simulink model "Template_v5_0_0_2026a_Original"  (R2026a)
settings: Solver=ode4  StopTime=tsim  FixedStep=baseRate  RelTol=1e-6  AbsTol=1e-6
undefined symbols (not defined in the file or in its folder): baseRate, dataRate, DiscIntNeverNeededParam, F_thrusters_BLACK, F_thrusters_BLUE, F_thrusters_RED, home_states_BLACK, home_states_BLUE, home_states_RED, IBLACK, IBLUE, init_states_BLACK, init_states_BLUE, init_states_RED, IRED, K_BLACK, K_BLUE, K_RED, labConsoleIP, mBLACK, mBLUE, mRED, Phase0_End, Phase1_End, Phase2_End, Phase3_End, Phase3_SubPhase1_End, Phase3_SubPhase2_End, Phase3_SubPhase3_End, Phase3_SubPhase4_End, Phase4_End, Phase5_End, platformSelection, PWMFreq, serverRate, simMode, tableDamping_BLACK, tableDamping_BLUE, tableDamping_RED, tableSlope, thrust_decay_BLACK, thrust_decay_BLUE, thrust_decay_RED, thruster_dist2CG_BLACK, thruster_dist2CG_BLUE, thruster_dist2CG_RED, xLength, yLength
libraries: simulink x18, dspinverses x3, nvidiaCommlib x1
(part 7 of 7)

== matlab function Template_v5_0_0_2026a_Original/Thruster & Float Control Code/Change BLUE Behavior/Calculate Duty Cycle/MATLAB Function5 ==
  data: H_final output; u_desired input; duty_cycles output; x0 input; thruster_dist2CG_BLUE parameter; F_thrusters_BLUE parameter; max_iters parameter; tol parameter; thrust_decay_BLUE parameter
function [H_final, duty_cycles] = optimize_duty_cycle_with_decay( ...
    u_desired, x0, thruster_dist2CG_BLUE, F_thrusters_BLUE, max_iters, tol, thrust_decay_BLUE)
    %OPTIMIZE_DUTY_CYCLE_WITH_DECAY 
    %   Iteratively optimizes thruster duty cycles while updating thrust decay.
    %
    %   Inputs:
    %       u_desired           - Desired force/torque vector [Fx; Fy; M] (3x1)
    %       x0                  - Initial guess for duty cycles (8x1)
    %       thruster_dist2CG_BLUE- Distances of thrusters from CG (vector, mm)
    %       F_thrusters_BLUE     - Thrust of each thruster (8x1, N): calibrated
    %                             (Calibration tab) or nominal (all eight alike)
    %       max_iters           - Maximum optimization iterations
    %       tol                 - Convergence tolerance (on duty cycles)
    %       thrust_decay_BLUE    - Thrust lost per extra valve open at once: with n
    %                             open, each gives 1 - thrust_decay_BLUE*(n - 1) of
    %                             its thrust alone (thruster calibration, Together)
    %
    %   Outputs:
    %       H_final     - Final H-matrix including thrust decay (3x8)
    %       duty_cycles - Optimized duty cycles (8x1)
    %

    % ---------------------------
    % Initialization
    % ---------------------------
    num_thrusters      = length(x0); %#ok<NASGU> % reserved if needed later
    duty_cycles        = x0;                     % current solution
    thrust_decay_factor = ones(8, 1);            % initial decay (each thruster's share)
    prev_duty_cycles   = duty_cycles + 2*tol;    % force first iteration

    % ---------------------------
    % Iterative optimization
    % ---------------------------
    for iter = 1:max_iters
        % Build system matrix H with current decay factor
        H = MakeHWithDecay(thruster_dist2CG_BLUE, F_thrusters_BLUE, thrust_decay_factor);

        % Solve constrained least squares (box constraints: 0 ≤ x ≤ 1)
        duty_cycles = custom_constrained_least_squares(H, u_desired, duty_cycles);

        % Update each thruster's decay from the current duty cycles
        [thrust_decay_factor, ~] = check_thrust_decay(duty_cycles, thrust_decay_BLUE);

        % Check convergence (∞-norm difference)
        if norm(duty_cycles - prev_duty_cycles, Inf) < tol
            H_final = MakeHWithDecayRecalculateForce(thruster_dist2CG_BLUE, F_thrusters_BLUE, thrust_decay_factor);
            return;
        end

        % Update reference for next iteration
        prev_duty_cycles = duty_cycles;
    end

    % If not converged within max_iters, return final H with last decay
    H_final = MakeHWithDecayRecalculateForce(thruster_dist2CG_BLUE, F_thrusters_BLUE, thrust_decay_factor);
end


% ========================================================================
% Custom Constrained Least Squares Solver
% ========================================================================
function x_opt = custom_constrained_least_squares(H, b, x0)
    %CUSTOM_CONSTRAINED_LEAST_SQUARES
    %   Solves min_x ||H*x - b||^2 subject to 0 <= x <= 1
    %   using projected gradient descent with backtracking line search.
    %
    %   Inputs:
    %       H   - System matrix (3x8)
    %       b   - Desired vector (3x1)
    %       x0  - Initial guess (8x1)
    %
    %   Output:
    %       x_opt - Optimal duty cycle vector (8x1)

    % Parameters
    max_iterations = 100;
    tolerance      = 1e-6;
    alpha          = 0.01;  % initial step size
    beta           = 0.5;   % backtracking factor

    % Initialization
    x      = x0;
    x_prev = x0 + 2*tolerance;

    % Precompute matrices
    HtH = H' * H;
    Htb = H' * b;

    for iter = 1:max_iterations
        % Gradient of ||H*x - b||^2
        gradient = 2 * (HtH*x - Htb);

        % Store objective for comparison
        current_obj = norm(H*x - b)^2;

        % Backtracking line search
        step_size = alpha;
        for ls_iter = 1:20
            x_new = x - step_size * gradient;
            x_new = max(0, min(1, x_new)); % project into [0,1]

            new_obj = norm(H*x_new - b)^2;
            if new_obj < current_obj
                break; % accept step
            else
                step_size = step_size * beta;
            end
        end

        % Update
        x = x_new;

        % Convergence check
        if norm(x - x_prev) < tolerance
            break;
        end

        % Adaptive step size tuning
        if iter > 1 && new_obj < current_obj
            alpha = min(alpha * 1.1, 0.1); % speed up if progress
        else
            alpha = alpha * 0.9;           % slow down otherwise
        end

        % Store for next iteration
        x_prev = x;
    end

    x_opt = x;
end


% ========================================================================
% Construct H-matrix (with decay factor)
% ========================================================================
function H = MakeHWithDecay(thruster_dist2CG, F_thrusters, thrust_decay_factor)
    %MAKEHWITHDECAY
    %   Builds the H matrix that maps thruster duty cycles to [Fx; Fy; M],
    %   applying each thruster's thrust decay (8x1, or one for all).
    %
    %   Outputs H as (3x8)

    % Convert thruster arm distances to meters
    adjusted_dist = thruster_dist2CG / 1000;

    % Thruster directions (X, Y, and moment arm)
    Vec1 = [-1; -1;  0;  0;  1;  1;  0;  0]; % X
    Vec2 = [ 0;  0;  1;  1;  0;  0; -1; -1]; % Y
    Vec3 = adjusted_dist;                    % moment (Z)

    Mat1 = [Vec1, Vec2, Vec3]';

    % Thruster forces (scaled by decay)
    F_decayed = F_thrusters(:) .* thrust_decay_factor(:);

    % Build diagonal scaling
    Mat2 = diag(F_decayed / 2);

    % Final mapping
    H = Mat1 * Mat2;
end


% ========================================================================
% Construct H-matrix (recalculate full force with decay)
% ========================================================================
function H = MakeHWithDecayRecalculateForce(thruster_dist2CG, F_thrusters, thrust_decay_factor)
    %MAKEHWITHDECAYRECALCULATEFORCE
    %   Same as MakeHWithDecay but applies full nominal force scaling.

    adjusted_dist = thruster_dist2CG / 1000;

    Vec1 = [-1; -1;  0;  0;  1;  1;  0;  0];
    Vec2 = [ 0;  0;  1;  1;  0;  0; -1; -1];
    Vec3 = adjusted_dist;

    Mat1 = [Vec1, Vec2, Vec3]';

    F_decayed = F_thrusters(:) .* thrust_decay_factor(:);

    Mat2 = diag(F_decayed);

    H = Mat1 * Mat2;
end


% ========================================================================
% Thrust Decay Update Rule
% ========================================================================
function [thrust_decay_factor, count] = check_thrust_decay(PWMs, decay_per_valve)
    %CHECK_THRUST_DECAY
    %   Each thruster's share of its thrust alone over one PWM period. The
    %   valves share one regulated supply: with n open at once, each gives
    %   max(0, 1 - decay_per_valve*(n - 1)) of its thrust alone (linear, as
    %   the thruster calibration's Together stage measures it). The Teensy
    %   opens every valve at the start of each PWM period and closes each
    %   after its duty cycle, so between two closings the number open is
    %   known, and each thruster's share is the average over its own opening.
    %
    %   Inputs:
    %       PWMs            - Duty cycle vector (8x1)
    %       decay_per_valve - Thrust lost per extra valve open (scalar)
    %
    %   Outputs:
    %       thrust_decay_factor - Each thruster's share of its thrust (8x1)
    %       count               - Number of active thrusters

    % Normalize if needed
    if max(PWMs) > 1
        PWMs = PWMs / max(PWMs);
    end
    duty = max(PWMs(:), 0);

    % Active thrusters
    count = sum(duty > 0);

    % The instants the valves close, in order
    closing = sort(duty);

    thrust_decay_factor = ones(8, 1);
    for i = 1:8
        if duty(i) > 0
            share = 0;
            t0 = 0;
            for k = 1:8
                t1 = min(closing(k), duty(i));
                if t1 > t0
                    n_open = sum(duty >= t1);   % valves open from t0 to t1
                    share = share + (t1 - t0) * max(0, 1 - decay_per_valve*(n_open - 1));
                    t0 = t1;
                end
            end
            thrust_decay_factor(i) = share / duty(i);
        end
    end
end

== matlab function Template_v5_0_0_2026a_Original/Thruster & Float Control Code/Change BLUE Behavior/Calculate Duty Cycle/MATLAB Function1 ==
  data: ThrustPer_Final output; ThrustPer input; PWMFreq parameter
function ThrustPer_Final  = ThrusterSat(ThrustPer, PWMFreq)

    ValveTime       = 0.007;
    TControl        = 1/PWMFreq;

    ThrustPer_Final = zeros(8,1);
    
    if max(ThrustPer) > 1
        ThrustPer_Sat = ThrustPer/max(ThrustPer);
    else
        ThrustPer_Sat = ThrustPer;
    end
    
    for i = 1:8
        if ThrustPer_Sat(i) > ValveTime/TControl 
            ThrustPer_Final(i) = ThrustPer_Sat(i);
        else
            ThrustPer_Final(i) = 0;
        end
    end


end

== matlab function Template_v5_0_0_2026a_Original/PhaseSpace Camera Code/Use Hardware to Obtain States/Store RED Data/Subsystem2/Enabled Subsystem/MATLAB Function ==
  data: y input; dy output; dt input; tau input; ema_prev input; ema output
function [dy, ema] = realtime_derivative_ema(y, dt, tau, ema_prev)
    % Compute smoothed derivative using Exponential Moving Average
    %
    % Inputs:
    %   y        : Current measurement
    %   dt       : Time step
    %   tau      : Time constant for EMA filter (larger = more smoothing)
    %   ema_prev : Previous EMA value
    %
    % Outputs:
    %   dy  : Smoothed derivative estimate
    %   ema : Updated EMA value
    
    % Calculate smoothing factor from time constant
    alpha = 1 - exp(-dt ./ tau);
    
    % Update Exponential Moving Average
    ema = alpha .* y + (1 - alpha) .* ema_prev;
    
    % Compute derivative using finite difference on smoothed values
    dy = (ema - ema_prev) ./ dt;
end

== matlab function Template_v5_0_0_2026a_Original/PhaseSpace Camera Code/Use Hardware to Obtain States/Store BLACK Data/Calculate True Time Step/MATLAB Function ==
  data: dt input; dt_out output; dataRate input
function dt_out = CheckforInvalidTime(dt, dataRate)

    if dt <= 0

        dt_out = dataRate;

    else

        dt_out = dt;

    end


end

== matlab function Template_v5_0_0_2026a_Original/PhaseSpace Camera Code/Use Hardware to Obtain States/Store RED Data/Calculate True Time Step/MATLAB Function ==
  data: dt input; dt_out output; dataRate input
function dt_out = CheckforInvalidTime(dt, dataRate)

    if dt <= 0

        dt_out = dataRate;

    else

        dt_out = dt;

    end


end

== matlab function Template_v5_0_0_2026a_Original/PhaseSpace Camera Code/Use Hardware to Obtain States/Store BLACK Data/Subsystem1/Enabled Subsystem/MATLAB Function ==
  data: y input; dy output; dt input; tau input; ema_prev input; ema output
function [dy, ema] = realtime_derivative_ema(y, dt, tau, ema_prev)
    % Compute smoothed derivative using Exponential Moving Average
    %
    % Inputs:
    %   y        : Current measurement
    %   dt       : Time step
    %   tau      : Time constant for EMA filter (larger = more smoothing)
    %   ema_prev : Previous EMA value
    %
    % Outputs:
    %   dy  : Smoothed derivative estimate
    %   ema : Updated EMA value
    
    % Calculate smoothing factor from time constant
    alpha = 1 - exp(-dt ./ tau);
    
    % Update Exponential Moving Average
    ema = alpha .* y + (1 - alpha) .* ema_prev;
    
    % Compute derivative using finite difference on smoothed values
    dy = (ema - ema_prev) ./ dt;
end

== matlab function Template_v5_0_0_2026a_Original/PhaseSpace Camera Code/Use Hardware to Obtain States/Store BLACK Data/Subsystem2/Enabled Subsystem/MATLAB Function ==
  data: y input; dy output; dt input; tau input; ema_prev input; ema output
function [dy, ema] = realtime_derivative_ema(y, dt, tau, ema_prev)
    % Compute smoothed derivative using Exponential Moving Average
    %
    % Inputs:
    %   y        : Current measurement
    %   dt       : Time step
    %   tau      : Time constant for EMA filter (larger = more smoothing)
    %   ema_prev : Previous EMA value
    %
    % Outputs:
    %   dy  : Smoothed derivative estimate
    %   ema : Updated EMA value
    
    % Calculate smoothing factor from time constant
    alpha = 1 - exp(-dt ./ tau);
    
    % Update Exponential Moving Average
    ema = alpha .* y + (1 - alpha) .* ema_prev;
    
    % Compute derivative using finite difference on smoothed values
    dy = (ema - ema_prev) ./ dt;
end

== matlab function Template_v5_0_0_2026a_Original/PhaseSpace Camera Code/Use Hardware to Obtain States/Store BLUE Data/Calculate True Time Step/MATLAB Function ==
  data: dt input; dt_out output; dataRate input
function dt_out = CheckforInvalidTime(dt, dataRate)

    if dt <= 0

        dt_out = dataRate;

    else

        dt_out = dt;

    end


end

== matlab function Template_v5_0_0_2026a_Original/PhaseSpace Camera Code/Use Hardware to Obtain States/Store BLUE Data/Subsystem1/Enabled Subsystem/MATLAB Function ==
  data: y input; dy output; dt input; tau input; ema_prev input; ema output
function [dy, ema] = realtime_derivative_ema(y, dt, tau, ema_prev)
    % Compute smoothed derivative using Exponential Moving Average
    %
    % Inputs:
    %   y        : Current measurement
    %   dt       : Time step
    %   tau      : Time constant for EMA filter (larger = more smoothing)
    %   ema_prev : Previous EMA value
    %
    % Outputs:
    %   dy  : Smoothed derivative estimate
    %   ema : Updated EMA value
    
    % Calculate smoothing factor from time constant
    alpha = 1 - exp(-dt ./ tau);
    
    % Update Exponential Moving Average
    ema = alpha .* y + (1 - alpha) .* ema_prev;
    
    % Compute derivative using finite difference on smoothed values
    dy = (ema - ema_prev) ./ dt;
end

== matlab function Template_v5_0_0_2026a_Original/PhaseSpace Camera Code/Use Hardware to Obtain States/Store BLUE Data/Subsystem2/Enabled Subsystem/MATLAB Function ==
  data: y input; dy output; dt input; tau input; ema_prev input; ema output
function [dy, ema] = realtime_derivative_ema(y, dt, tau, ema_prev)
    % Compute smoothed derivative using Exponential Moving Average
    %
    % Inputs:
    %   y        : Current measurement
    %   dt       : Time step
    %   tau      : Time constant for EMA filter (larger = more smoothing)
    %   ema_prev : Previous EMA value
    %
    % Outputs:
    %   dy  : Smoothed derivative estimate
    %   ema : Updated EMA value
    
    % Calculate smoothing factor from time constant
    alpha = 1 - exp(-dt ./ tau);
    
    % Update Exponential Moving Average
    ema = alpha .* y + (1 - alpha) .* ema_prev;
    
    % Compute derivative using finite difference on smoothed values
    dy = (ema - ema_prev) ./ dt;
end

== matlab function Template_v5_0_0_2026a_Original/Data Logger Subsystem/Data Logger/MATLAB Function ==
  data: Input input; inputSize output
function inputSize = getSizeInput(Input)

    inputSize = max(size(Input));

end

== matlab function Template_v5_0_0_2026a_Original/Simulate Plant Dynamics/RED and ARM Dynamics/RED Only/Dynamics Model for RED/MATLAB Function ==
  data: control_inputs input; position input; velocity input; floating input; x_ddot output; mRED parameter; IRED parameter; tableSlope parameter; tableDamping_RED parameter

    function x_ddot = RED_dynamics(control_inputs, position, velocity, floating, mRED, IRED, tableSlope, tableDamping_RED)

        %#codegen
        % Fully define the size of x_ddot() for code generation:
        x_ddot     = zeros(3,1);

        % Extract the servicer model parameters from the model_param vector defined
        % in initialize.m:

        % Extract the control inputs from the control_input vector:
        Fx        = control_inputs(1);              % [N]
        Fy        = control_inputs(2);              % [N]
        Tz        = control_inputs(3);              % [N.m]

        % Calculate the state acceleration vector:
        x_ddot(1) = Fx/mRED;                      % [m/s^2]
        x_ddot(2) = Fy/mRED;                      % [m/s^2]
        x_ddot(3) = Tz/IRED;                      % [rad/s^2]
% The table's pull (the Calibration tab; spot.dynamics.tableSlope): while the platform floats
% (FLOATING: Float_State), it slides down the table's slope and its air bearings drag it. POSITION
% and VELOCITY are the previous step's (Previous Position, Previous Velocity). tableSlope is all
% zeros on a level table (Scenario: Table Slope off, or no calibration).
if floating ~= 0
    x_ddot(1:2) = x_ddot(1:2) + spot.dynamics.tableSlope(position, velocity, tableSlope, tableDamping_RED);
end


    end

== matlab function Template_v5_0_0_2026a_Original/Check Connection/Change BLACK Behavior/UDP Send ==
  data: data input
function sendHeartbeat(data)
%SENDHEARTBEAT A heartbeat (int32) showing that this platform's program is running.
%   Sends data to 255.255.255.255:33002 every step (was a UDP Send block; see help
%   spot.hardware.udpSend).
%#codegen
spot.hardware.udpSend('255.255.255.255', 33002, data);
end

== matlab function Template_v5_0_0_2026a_Original/Check Connection/Change BLUE Behavior/UDP Send ==
  data: data input
function sendHeartbeat(data)
%SENDHEARTBEAT A heartbeat (int32) showing that this platform's program is running.
%   Sends data to 255.255.255.255:33003 every step (was a UDP Send block; see help
%   spot.hardware.udpSend).
%#codegen
spot.hardware.udpSend('255.255.255.255', 33003, data);
end

== matlab function Template_v5_0_0_2026a_Original/Simulate Plant Dynamics/RED and ARM Dynamics/RED + ARM/Calculated & Store Measured States/Subsystem5/Enabled Subsystem/MATLAB Function ==
  data: y input; dy output; dt input; tau input; ema_prev input; ema output
function [dy, ema] = realtime_derivative_ema(y, dt, tau, ema_prev)
    % Compute smoothed derivative using Exponential Moving Average
    %
    % Inputs:
    %   y        : Current measurement
    %   dt       : Time step
    %   tau      : Time constant for EMA filter (larger = more smoothing)
    %   ema_prev : Previous EMA value
    %
    % Outputs:
    %   dy  : Smoothed derivative estimate
    %   ema : Updated EMA value
    
    % Calculate smoothing factor from time constant
    alpha = 1 - exp(-dt ./ tau);
    
    % Update Exponential Moving Average
    ema = alpha .* y + (1 - alpha) .* ema_prev;
    
    % Compute derivative using finite difference on smoothed values
    dy = (ema - ema_prev) ./ dt;
end

== matlab function Template_v5_0_0_2026a_Original/Simulate Plant Dynamics/RED and ARM Dynamics/RED + ARM/Data @ Measurement Rate/Calculate True Time Step/MATLAB Function ==
  data: dt input; dt_out output; dataRate input
function dt_out = CheckforInvalidTime(dt, dataRate)

    if dt <= 0

        dt_out = dataRate;

    else

        dt_out = dt;

    end


end

== matlab function Template_v5_0_0_2026a_Original/PhaseSpace Camera Code/Use Hardware to Obtain States/Receive and Process Phasespace Data/Receive PhaseSpace Data ==
  data: packet output; newPackets output; age output; labConsoleIP parameter
function [packet, newPackets, age] = receivePhaseSpaceData(labConsoleIP)
%RECEIVEPHASESPACEDATA The newest PhaseSpace packet from the lab console (TX2), every step.
%   packet: 115 values (positions, velocities, LEDs and, during an experiment, the experiment
%   clock); newPackets: packets since the last step; age: seconds since it arrived (-1 = none
%   yet). See help spot.hardware.phasespaceLatest.
%#codegen
[packet, newPackets, age] = spot.hardware.phasespaceLatest(31534, labConsoleIP);
end

== matlab function Template_v5_0_0_2026a_Original/Check Connection/Change RED Behavior/UDP Send ==
  data: data input
function sendHeartbeat(data)
%SENDHEARTBEAT A heartbeat (int32) showing that this platform's program is running.
%   Sends data to 255.255.255.255:33001 every step (was a UDP Send block; see help
%   spot.hardware.udpSend).
%#codegen
spot.hardware.udpSend('255.255.255.255', 33001, data);
end

== matlab function Template_v5_0_0_2026a_Original/4 - Control/Default LQR Control (BLACK)/Calculate Error/MATLAB Function ==
  data: Rz_path input; Rz_error output; Rz_measured input
function Rz_error = SmoothAngularDifference(Rz_path, Rz_measured)

    Rz_error = mod(Rz_measured-Rz_path+pi, 2*pi)-pi;


end

== matlab function Template_v5_0_0_2026a_Original/PhaseSpace Camera Code/Use Hardware to Obtain States/Receive and Process Phasespace Data/Experiment Clock/Send Sync. Time/Change BLACK Behavior/UDP Send (GUI) ==
  data: data input; labConsoleIP parameter
function sendExperimentTime(data, labConsoleIP)
%SENDEXPERIMENTTIME This platform's experiment time, to the lab console (its Experiment tab).
%   Sends data to the lab console (labConsoleIP):48721 every step (was a UDP Send block; see help
%   spot.hardware.udpSend).
%#codegen
spot.hardware.udpSend(labConsoleIP, 48721, data);
end

== matlab function Template_v5_0_0_2026a_Original/PhaseSpace Camera Code/Use Hardware to Obtain States/Receive and Process Phasespace Data/Experiment Clock/Send Sync. Time/Change BLUE Behavior/UDP Send (GUI) ==
  data: data input; labConsoleIP parameter
function sendExperimentTime(data, labConsoleIP)
%SENDEXPERIMENTTIME This platform's experiment time, to the lab console (its Experiment tab).
%   Sends data to the lab console (labConsoleIP):48722 every step (was a UDP Send block; see help
%   spot.hardware.udpSend).
%#codegen
spot.hardware.udpSend(labConsoleIP, 48722, data);
end

== matlab function Template_v5_0_0_2026a_Original/PhaseSpace Camera Code/Use Hardware to Obtain States/Receive and Process Phasespace Data/Experiment Clock/Send Sync. Time/Change RED Behavior/UDP Send (GUI) ==
  data: data input; labConsoleIP parameter
function sendExperimentTime(data, labConsoleIP)
%SENDEXPERIMENTTIME This platform's experiment time, to the lab console (its Experiment tab).
%   Sends data to the lab console (labConsoleIP):48720 every step (was a UDP Send block; see help
%   spot.hardware.udpSend).
%#codegen
spot.hardware.udpSend(labConsoleIP, 48720, data);
end

== matlab function Template_v5_0_0_2026a_Original/Receive Data from Orin/Subsystem/UDP Receive ==
  data: data output; newPackets output; age output
function [data, newPackets, age] = receiveFromOrin()
%RECEIVEFROMORIN The newest states and confidence from the Orin (vision computer).
%   The newest packet on UDP 36845 (was a UDP Receive block): data, the packets since the
%   last step, and its age [s] (-1 = none yet). See help spot.hardware.udpReceive.
%#codegen
[data, newPackets, age] = spot.hardware.udpReceive(36845, '0.0.0.0', 4, 'single');
end

== matlab function Template_v5_0_0_2026a_Original/Send Data to Orin/Subsystem/UDP Send ==
  data: data input
function sendStatesToOrin(data)
%SENDSTATESTOORIN The experiment time and the platforms' states, to the Orin (vision computer).
%   Sends data to 192.168.1.115:46875 every step (was a UDP Send block; see help
%   spot.hardware.udpSend).
%#codegen
spot.hardware.udpSend('192.168.1.115', 46875, data);
end

== matlab function Template_v5_0_0_2026a_Original/Live Data Streams/Live Stream 4/Stream ==
  data: u input; t input; whoAmI input; isSim input; streamLabel parameter; labConsoleIP parameter
function streamData(u, t, whoAmI, isSim, streamLabel, labConsoleIP)
%STREAMDATA Sends this block's input to the SPOT Console's live plot, every step.
%   Its name in the plot is the name of what is connected (e.g. a Data Store Read's data store)
%   or the name typed into the block (double-click it). See help spot.hardware.liveStream.
%#codegen
spot.hardware.liveStream(streamLabel, t, u, whoAmI, isSim, labConsoleIP);
end

== matlab function Template_v5_0_0_2026a_Original/Thruster & Float Control Code/Change BLACK Behavior/Calculate Duty Cycle/Generate Initial Guess/MATLAB Function ==
  data: H output; thruster_dist2CG_BLACK parameter; F_thrusters_BLACK parameter
function H = MakeH(thruster_dist2CG_BLACK,F_thrusters_BLACK)

    Vec1 = [ -1
             -1
              0 
              0
              1
              1
              0
              0 ];
          
    Vec2 = [  0
              0
              1
              1
              0
              0
             -1
             -1 ];
         
    Vec3 = thruster_dist2CG_BLACK./1000;
    
    Mat1 = [Vec1, Vec2, Vec3]';
    
    Mat2 = diag((F_thrusters_BLACK./2));
    
    H    = Mat1*Mat2;

end

== matlab function Template_v5_0_0_2026a_Original/Thruster & Float Control Code/Change BLACK Behavior/Calculate Duty Cycle/Rotate Forces to Inertial/Create Rotation Matrix ==
  data: Rz input; C_Ib output
function C_Ib = RotateFrame(Rz)

C_bI = [  cos(Rz) sin(Rz)
         -sin(Rz) cos(Rz) ];

C_Ib = inv(C_bI);

end

== matlab function Template_v5_0_0_2026a_Original/Live Data Streams/Live Stream 2/Stream ==
  data: u input; t input; whoAmI input; isSim input; streamLabel parameter; labConsoleIP parameter
function streamData(u, t, whoAmI, isSim, streamLabel, labConsoleIP)
%STREAMDATA Sends this block's input to the SPOT Console's live plot, every step.
%   Its name in the plot is the name of what is connected (e.g. a Data Store Read's data store)
%   or the name typed into the block (double-click it). See help spot.hardware.liveStream.
%#codegen
spot.hardware.liveStream(streamLabel, t, u, whoAmI, isSim, labConsoleIP);
end

== matlab function Template_v5_0_0_2026a_Original/Live Data Streams/Live Stream 3/Stream ==
  data: u input; t input; whoAmI input; isSim input; streamLabel parameter; labConsoleIP parameter
function streamData(u, t, whoAmI, isSim, streamLabel, labConsoleIP)
%STREAMDATA Sends this block's input to the SPOT Console's live plot, every step.
%   Its name in the plot is the name of what is connected (e.g. a Data Store Read's data store)
%   or the name typed into the block (double-click it). See help spot.hardware.liveStream.
%#codegen
spot.hardware.liveStream(streamLabel, t, u, whoAmI, isSim, labConsoleIP);
end

== matlab function Template_v5_0_0_2026a_Original/4 - Control/Default LQR Control (RED)/Calculate Error/MATLAB Function ==
  data: Rz_path input; Rz_error output; Rz_measured input
function Rz_error = SmoothAngularDifference(Rz_path, Rz_measured)

    Rz_error = mod(Rz_measured-Rz_path+pi, 2*pi)-pi;


end

== matlab function Template_v5_0_0_2026a_Original/Thruster & Float Control Code/Change BLACK Behavior/Rotate Forces to Body/Create Rotation Matrix ==
  data: Rz input; C_bI output
function C_bI = RotateFrame(Rz)

C_bI = [  cos(Rz) sin(Rz)
         -sin(Rz) cos(Rz) ];

end

== matlab function Template_v5_0_0_2026a_Original/Thruster & Float Control Code/Change BLUE Behavior/Calculate Duty Cycle/Generate Initial Guess/MATLAB Function ==
  data: H output; thruster_dist2CG_BLUE parameter; F_thrusters_BLUE parameter
function H = MakeH(thruster_dist2CG_BLUE,F_thrusters_BLUE)

    Vec1 = [ -1
             -1
              0 
              0
              1
              1
              0
              0 ];
          
    Vec2 = [  0
              0
              1
              1
              0
              0
             -1
             -1 ];
         
    Vec3 = thruster_dist2CG_BLUE./1000;
    
    Mat1 = [Vec1, Vec2, Vec3]';
    
    Mat2 = diag((F_thrusters_BLUE./2));
    
    H    = Mat1*Mat2;

end

== matlab function Template_v5_0_0_2026a_Original/Thruster & Float Control Code/Change BLUE Behavior/Calculate Duty Cycle/Rotate Forces to Inertial/Create Rotation Matrix ==
  data: Rz input; C_Ib output
function C_Ib = RotateFrame(Rz)

C_bI = [  cos(Rz) sin(Rz)
         -sin(Rz) cos(Rz) ];

C_Ib = inv(C_bI);

end

== matlab function Template_v5_0_0_2026a_Original/Thruster & Float Control Code/Change BLUE Behavior/Rotate Forces to Body/Create Rotation Matrix ==
  data: Rz input; C_bI output
function C_bI = RotateFrame(Rz)

C_bI = [  cos(Rz) sin(Rz)
         -sin(Rz) cos(Rz) ];

end

== matlab function Template_v5_0_0_2026a_Original/Thruster & Float Control Code/Change RED Behavior/Calculate Duty Cycle/Generate Initial Guess/MATLAB Function ==
  data: H output; thruster_dist2CG_RED parameter; F_thrusters_RED parameter
function H = MakeH(thruster_dist2CG_RED,F_thrusters_RED)

    Vec1 = [ -1
             -1
              0 
              0
              1
              1
              0
              0 ];
          
    Vec2 = [  0
              0
              1
              1
              0
              0
             -1
             -1 ];
         
    Vec3 = thruster_dist2CG_RED./1000;
    
    Mat1 = [Vec1, Vec2, Vec3]';
    
    Mat2 = diag((F_thrusters_RED./2));
    
    H    = Mat1*Mat2;

end

== matlab function Template_v5_0_0_2026a_Original/Thruster & Float Control Code/Change RED Behavior/Calculate Duty Cycle/MATLAB Function5 ==
  data: H_final output; u_desired input; duty_cycles output; x0 input; thruster_dist2CG_RED parameter; F_thrusters_RED parameter; max_iters parameter; tol parameter; thrust_decay_RED parameter
function [H_final, duty_cycles] = optimize_duty_cycle_with_decay( ...
    u_desired, x0, thruster_dist2CG_RED, F_thrusters_RED, max_iters, tol, thrust_decay_RED)
    %OPTIMIZE_DUTY_CYCLE_WITH_DECAY 
    %   Iteratively optimizes thruster duty cycles while updating thrust decay.
    %
    %   Inputs:
    %       u_desired           - Desired force/torque vector [Fx; Fy; M] (3x1)
    %       x0                  - Initial guess for duty cycles (8x1)
    %       thruster_dist2CG_RED- Distances of thrusters from CG (vector, mm)
    %       F_thrusters_RED     - Thrust of each thruster (8x1, N): calibrated
    %                             (Calibration tab) or nominal (all eight alike)
    %       max_iters           - Maximum optimization iterations
    %       tol                 - Convergence tolerance (on duty cycles)
    %       thrust_decay_RED    - Thrust lost per extra valve open at once: with n
    %                             open, each gives 1 - thrust_decay_RED*(n - 1) of
    %                             its thrust alone (thruster calibration, Together)
    %
    %   Outputs:
    %       H_final     - Final H-matrix including thrust decay (3x8)
    %       duty_cycles - Optimized duty cycles (8x1)
    %

    % ---------------------------
    % Initialization
    % ---------------------------
    num_thrusters      = length(x0); %#ok<NASGU> % reserved if needed later
    duty_cycles        = x0;                     % current solution
    thrust_decay_factor = ones(8, 1);            % initial decay (each thruster's share)
    prev_duty_cycles   = duty_cycles + 2*tol;    % force first iteration

    % ---------------------------
    % Iterative optimization
    % ---------------------------
    for iter = 1:max_iters
        % Build system matrix H with current decay factor
        H = MakeHWithDecay(thruster_dist2CG_RED, F_thrusters_RED, thrust_decay_factor);

        % Solve constrained least squares (box constraints: 0 ≤ x ≤ 1)
        duty_cycles = custom_constrained_least_squares(H, u_desired, duty_cycles);

        % Update each thruster's decay from the current duty cycles
        [thrust_decay_factor, ~] = check_thrust_decay(duty_cycles, thrust_decay_RED);

        % Check convergence (∞-norm difference)
        if norm(duty_cycles - prev_duty_cycles, Inf) < tol
            H_final = MakeHWithDecayRecalculateForce(thruster_dist2CG_RED, F_thrusters_RED, thrust_decay_factor);
            return;
        end

        % Update reference for next iteration
        prev_duty_cycles = duty_cycles;
    end

    % If not converged within max_iters, return final H with last decay
    H_final = MakeHWithDecayRecalculateForce(thruster_dist2CG_RED, F_thrusters_RED, thrust_decay_factor);
end


% ========================================================================
% Custom Constrained Least Squares Solver
% ========================================================================
function x_opt = custom_constrained_least_squares(H, b, x0)
    %CUSTOM_CONSTRAINED_LEAST_SQUARES
    %   Solves min_x ||H*x - b||^2 subject to 0 <= x <= 1
    %   using projected gradient descent with backtracking line search.
    %
    %   Inputs:
    %       H   - System matrix (3x8)
    %       b   - Desired vector (3x1)
    %       x0  - Initial guess (8x1)
    %
    %   Output:
    %       x_opt - Optimal duty cycle vector (8x1)

    % Parameters
    max_iterations = 100;
    tolerance      = 1e-6;
    alpha          = 0.01;  % initial step size
    beta           = 0.5;   % backtracking factor

    % Initialization
    x      = x0;
    x_prev = x0 + 2*tolerance;

    % Precompute matrices
    HtH = H' * H;
    Htb = H' * b;

    for iter = 1:max_iterations
        % Gradient of ||H*x - b||^2
        gradient = 2 * (HtH*x - Htb);

        % Store objective for comparison
        current_obj = norm(H*x - b)^2;

        % Backtracking line search
        step_size = alpha;
        for ls_iter = 1:20
            x_new = x - step_size * gradient;
            x_new = max(0, min(1, x_new)); % project into [0,1]

            new_obj = norm(H*x_new - b)^2;
            if new_obj < current_obj
                break; % accept step
            else
                step_size = step_size * beta;
            end
        end

        % Update
        x = x_new;

        % Convergence check
        if norm(x - x_prev) < tolerance
            break;
        end

        % Adaptive step size tuning
        if iter > 1 && new_obj < current_obj
            alpha = min(alpha * 1.1, 0.1); % speed up if progress
        else
            alpha = alpha * 0.9;           % slow down otherwise
        end

        % Store for next iteration
        x_prev = x;
    end

    x_opt = x;
end


% ========================================================================
% Construct H-matrix (with decay factor)
% ========================================================================
function H = MakeHWithDecay(thruster_dist2CG, F_thrusters, thrust_decay_factor)
    %MAKEHWITHDECAY
    %   Builds the H matrix that maps thruster duty cycles to [Fx; Fy; M],
    %   applying each thruster's thrust decay (8x1, or one for all).
    %
    %   Outputs H as (3x8)

    % Convert thruster arm distances to meters
    adjusted_dist = thruster_dist2CG / 1000;

    % Thruster directions (X, Y, and moment arm)
    Vec1 = [-1; -1;  0;  0;  1;  1;  0;  0]; % X
    Vec2 = [ 0;  0;  1;  1;  0;  0; -1; -1]; % Y
    Vec3 = adjusted_dist;                    % moment (Z)

    Mat1 = [Vec1, Vec2, Vec3]';

    % Thruster forces (scaled by decay)
    F_decayed = F_thrusters(:) .* thrust_decay_factor(:);

    % Build diagonal scaling
    Mat2 = diag(F_decayed / 2);

    % Final mapping
    H = Mat1 * Mat2;
end


% ========================================================================
% Construct H-matrix (recalculate full force with decay)
% ========================================================================
function H = MakeHWithDecayRecalculateForce(thruster_dist2CG, F_thrusters, thrust_decay_factor)
    %MAKEHWITHDECAYRECALCULATEFORCE
    %   Same as MakeHWithDecay but applies full nominal force scaling.

    adjusted_dist = thruster_dist2CG / 1000;

    Vec1 = [-1; -1;  0;  0;  1;  1;  0;  0];
    Vec2 = [ 0;  0;  1;  1;  0;  0; -1; -1];
    Vec3 = adjusted_dist;

    Mat1 = [Vec1, Vec2, Vec3]';

    F_decayed = F_thrusters(:) .* thrust_decay_factor(:);

    Mat2 = diag(F_decayed);

    H = Mat1 * Mat2;
end


% ========================================================================
% Thrust Decay Update Rule
% ========================================================================
function [thrust_decay_factor, count] = check_thrust_decay(PWMs, decay_per_valve)
    %CHECK_THRUST_DECAY
    %   Each thruster's share of its thrust alone over one PWM period. The
    %   valves share one regulated supply: with n open at once, each gives
    %   max(0, 1 - decay_per_valve*(n - 1)) of its thrust alone (linear, as
    %   the thruster calibration's Together stage measures it). The Teensy
    %   opens every valve at the start of each PWM period and closes each
    %   after its duty cycle, so between two closings the number open is
    %   known, and each thruster's share is the average over its own opening.
    %
    %   Inputs:
    %       PWMs            - Duty cycle vector (8x1)
    %       decay_per_valve - Thrust lost per extra valve open (scalar)
    %
    %   Outputs:
    %       thrust_decay_factor - Each thruster's share of its thrust (8x1)
    %       count               - Number of active thrusters

    % Normalize if needed
    if max(PWMs) > 1
        PWMs = PWMs / max(PWMs);
    end
    duty = max(PWMs(:), 0);

    % Active thrusters
    count = sum(duty > 0);

    % The instants the valves close, in order
    closing = sort(duty);

    thrust_decay_factor = ones(8, 1);
    for i = 1:8
        if duty(i) > 0
            share = 0;
            t0 = 0;
            for k = 1:8
                t1 = min(closing(k), duty(i));
                if t1 > t0
                    n_open = sum(duty >= t1);   % valves open from t0 to t1
                    share = share + (t1 - t0) * max(0, 1 - decay_per_valve*(n_open - 1));
                    t0 = t1;
                end
            end
            thrust_decay_factor(i) = share / duty(i);
        end
    end
end

== matlab function Template_v5_0_0_2026a_Original/Thruster & Float Control Code/Change RED Behavior/Calculate Duty Cycle/Rotate Forces to Inertial/Create Rotation Matrix ==
  data: Rz input; C_Ib output
function C_Ib = RotateFrame(Rz)

C_bI = [  cos(Rz) sin(Rz)
         -sin(Rz) cos(Rz) ];

C_Ib = inv(C_bI);

end

== matlab function Template_v5_0_0_2026a_Original/Thruster & Float Control Code/Change RED Behavior/Rotate Forces to Body/Create Rotation Matrix ==
  data: Rz input; C_bI output
function C_bI = RotateFrame(Rz)

C_bI = [  cos(Rz) sin(Rz)
         -sin(Rz) cos(Rz) ];

end

== matlab function Template_v5_0_0_2026a_Original/Thruster & Float Control Code/Change BLACK Behavior/Calculate Duty Cycle/MATLAB Function1 ==
  data: ThrustPer_Final output; ThrustPer input; PWMFreq parameter
function ThrustPer_Final  = ThrusterSat(ThrustPer, PWMFreq)

    ValveTime       = 0.007;
    TControl        = 1/PWMFreq;

    ThrustPer_Final = zeros(8,1);
    
    if max(ThrustPer) > 1
        ThrustPer_Sat = ThrustPer/max(ThrustPer);
    else
        ThrustPer_Sat = ThrustPer;
    end
    
    for i = 1:8
        if ThrustPer_Sat(i) > ValveTime/TControl 
            ThrustPer_Final(i) = ThrustPer_Sat(i);
        else
            ThrustPer_Final(i) = 0;
        end
    end


end

== matlab function Template_v5_0_0_2026a_Original/Thruster & Float Control Code/Change RED Behavior/Calculate Duty Cycle/MATLAB Function8 ==
  data: ThrustPer_Final output; ThrustPer input; PWMFreq parameter
function ThrustPer_Final  = ThrusterSat(ThrustPer, PWMFreq)

    ValveTime       = 0.007;
    TControl        = 1/PWMFreq;

    ThrustPer_Final = zeros(8,1);
    
    if max(ThrustPer) > 1
        ThrustPer_Sat = ThrustPer/max(ThrustPer);
    else
        ThrustPer_Sat = ThrustPer;
    end
    
    for i = 1:8
        if ThrustPer_Sat(i) > ValveTime/TControl 
            ThrustPer_Final(i) = ThrustPer_Sat(i);
        else
            ThrustPer_Final(i) = 0;
        end
    end


end

== matlab function Template_v5_0_0_2026a_Original/PhaseSpace Camera Code/Use Hardware to Obtain States/Receive and Process Phasespace Data/Experiment Clock/Experiment Time ==
  data: packet input; t output; age input; state output
function [t, state] = experimentClock(packet, age)
%EXPERIMENTCLOCK The experiment time from the PhaseSpace stream, the same on every platform.
%   t is 0 until the lab console's agreed start, then the shared clock [s]. state: 0 waiting,
%   1 counting down, 2 running, 3 running on this computer's clock (the shared one was lost).
%   See help spot.hardware.experimentTime.
%#codegen
[t, state] = spot.hardware.experimentTime(packet, age);
end

== matlab function Template_v5_0_0_2026a_Original/4 - Control/Default LQR Control (BLUE)/Calculate Error/MATLAB Function ==
  data: Rz_path input; Rz_error output; Rz_measured input
function Rz_error = SmoothAngularDifference(Rz_path, Rz_measured)

    Rz_error = mod(Rz_measured-Rz_path+pi, 2*pi)-pi;


end

== matlab function Template_v5_0_0_2026a_Original/Debugger/Send Debug Messages ==
  data: whoAmI input; isSim input; t input; red input; black input; blue input; labConsoleIP parameter
function sendDebugMessages(whoAmI, isSim, t, red, black, blue, labConsoleIP)
%SENDDEBUGMESSAGES Each platform's debug message, for the SPOT Console's Messages panel.
%   The texts in RED_Logger, BLACK_Logger and BLUE_Logger: on a platform, its own message goes
%   to the lab console (UDP 55001-55003, when it changes and every 0.5 s); in a simulation,
%   every change is recorded for the console. See help spot.hardware.debugMessages.
%#codegen
spot.hardware.debugMessages(whoAmI, isSim, t, red, black, blue, labConsoleIP);
end

== matlab function Template_v5_0_0_2026a_Original/Simulate Plant Dynamics/RED and ARM Dynamics/RED + ARM/Calculated & Store Measured States/Subsystem3/Enabled Subsystem/MATLAB Function ==
  data: y input; dy output; dt input; tau input; ema_prev input; ema output
function [dy, ema] = realtime_derivative_ema(y, dt, tau, ema_prev)
    % Compute smoothed derivative using Exponential Moving Average
    %
    % Inputs:
    %   y        : Current measurement
    %   dt       : Time step
    %   tau      : Time constant for EMA filter (larger = more smoothing)
    %   ema_prev : Previous EMA value
    %
    % Outputs:
    %   dy  : Smoothed derivative estimate
    %   ema : Updated EMA value
    
    % Calculate smoothing factor from time constant
    alpha = 1 - exp(-dt ./ tau);
    
    % Update Exponential Moving Average
    ema = alpha .* y + (1 - alpha) .* ema_prev;
    
    % Compute derivative using finite difference on smoothed values
    dy = (ema - ema_prev) ./ dt;
end

== matlab function Template_v5_0_0_2026a_Original/Simulate Plant Dynamics/RED and ARM Dynamics/RED Only/Calculated & Store Measured States/Subsystem2/Enabled Subsystem/MATLAB Function ==
  data: y input; dy output; dt input; tau input; ema_prev input; ema output
function [dy, ema] = realtime_derivative_ema(y, dt, tau, ema_prev)
    % Compute smoothed derivative using Exponential Moving Average
    %
    % Inputs:
    %   y        : Current measurement
    %   dt       : Time step
    %   tau      : Time constant for EMA filter (larger = more smoothing)
    %   ema_prev : Previous EMA value
    %
    % Outputs:
    %   dy  : Smoothed derivative estimate
    %   ema : Updated EMA value
    
    % Calculate smoothing factor from time constant
    alpha = 1 - exp(-dt ./ tau);
    
    % Update Exponential Moving Average
    ema = alpha .* y + (1 - alpha) .* ema_prev;
    
    % Compute derivative using finite difference on smoothed values
    dy = (ema - ema_prev) ./ dt;
end
